simulink model "ecu_spdst"  (R2026a)
settings: Solver=FixedStepDiscrete  StopTime=10  FixedStep=0.001  SampleTimeConstraint=STIndependent
Description:
  | Speed states. Source of truth for firmware/gen/ecu_spdst.
settings Model: Creator=jj1001000  LastModifiedBy=jj1001000
settings OptimizationCC: DefaultUnderspecifiedDataType=single
settings DebuggingCC: ParameterPrecisionLossMsg=none
settings HardwareCC: ProdLargestAtomicInteger=Long  ProdLargestAtomicFloat=Double  ProdHWDeviceType=ARM Compatible->ARM Cortex-M
settings RTWCC: SystemTargetFile=ert.tlc  GenCodeOnly=on  Description=Embedded Coder
settings ERTTargetCC: UtilityFuncGeneration=Shared location  IncludeMdlTerminateFcn=off  CodeInterfacePackaging=Reusable function  SupportNonFinite=off

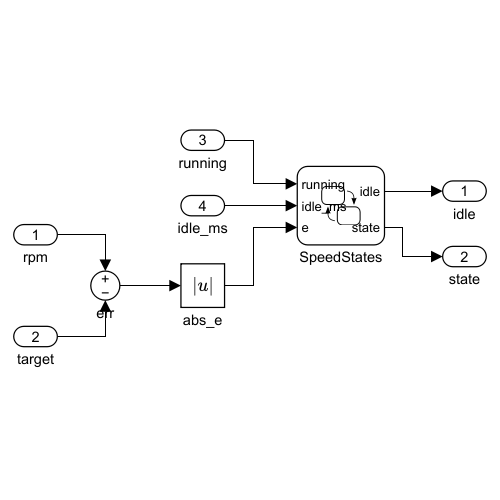
[thumbnail: Simulink's stored preview of the top-level diagram]
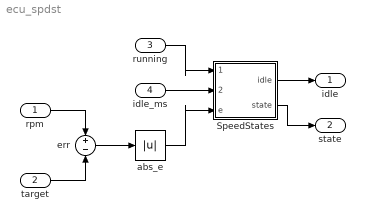
== system ecu_spdst ==
  rpm : Inport  OutDataTypeStr=single
  target : Inport  Port=2  OutDataTypeStr=single
  running : Inport  Port=3  OutDataTypeStr=uint8
  idle_ms : Inport  Port=4  OutDataTypeStr=uint32
  SpeedStates : Stateflow chart  TreatAsAtomicUnit=on
  abs_e : Abs  SaturateOnIntegerOverflow=off
  err : Sum  Inputs=+-
  idle : Outport  OutDataTypeStr=uint8
  state : Outport  Port=2  OutDataTypeStr=uint8
  wires:
  err/1 -> abs_e/1
  target/1 -> err/2
  rpm/1 -> err/1
  running/1 -> SpeedStates/1(running)
  SpeedStates/2(state) -> state/1
  SpeedStates/1(idle) -> idle/1
  idle_ms/1 -> SpeedStates/2(idle_ms)
  abs_e/1 -> SpeedStates/3(e)

== stateflow chart ecu_spdst/SpeedStates ==
  settings: updateMethod=DISCRETE  executeAtInitialization=1
  state OFF
    entry: idle = uint8(0); state = uint8(0);
  state IDLE
    entry: idle = uint8(1); state = uint8(1);
    during: n = n + uint32(1);
  state OPERATING
    entry: idle = uint8(0); state = uint8(2);
    during: if e <= single(15), n = n + uint32(1); else, n = uint32(0); end
  state STEADY
    entry: idle = uint8(0); state = uint8(3);
  (default) -> OFF : {n = uint32(0); idle = uint8(0); state = uint8(0);}
  OFF -> IDLE [order 1] : [running ~= 0 && idle_ms > uint32(0)]{n = uint32(0);}
  IDLE -> OFF [order 1] : [running == 0]{n = uint32(0);}
  OPERATING -> OFF [order 1] : [running == 0]{n = uint32(0);}
  STEADY -> OFF [order 1] : [running == 0]{n = uint32(0);}
  OFF -> OPERATING [order 2] : [running ~= 0]{n = uint32(0);}
  IDLE -> OPERATING [order 2] : [n + uint32(1) >= idle_ms]{n = uint32(0);}
  OPERATING -> STEADY [order 2] : [e <= single(15) && n + uint32(1) >= uint32(1000)]{n = uint32(0);}
  STEADY -> OPERATING [order 2] : [e > single(30)]{n = uint32(0);}
  data: running input uint8; idle_ms input uint32; idle output uint8; state output uint8; e input single; n local uint32
